simulink library "tof_lib"  (R2026a)
settings: Solver=VariableStepAuto
values from neighbouring files (symbols this model uses):
  fc_tofGain = Simulink.Parameter(1.00901);    fc_tofGain.CoderInfo.StorageClass      = 'ExportedGlobal'    [init_params.m]
  fc_tofIntercept = Simulink.Parameter(14.477);     fc_tofIntercept.CoderInfo.StorageClass = 'ExportedGlobal'    [init_params.m]
settings Model: Creator=Cyril Calo  LastModifiedBy=Cyril Calo

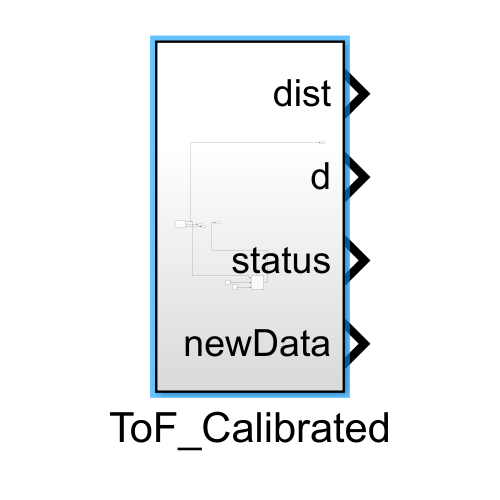
[thumbnail: Simulink's stored preview of the top-level diagram]
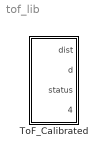
== system tof_lib ==
  ToF_Calibrated : Subsystem

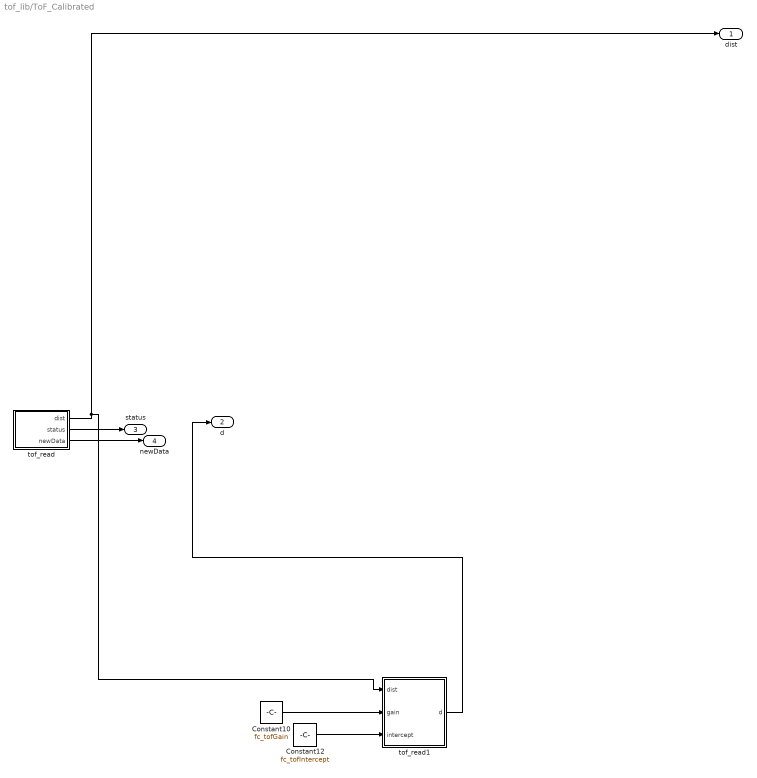
== system tof_lib/ToF_Calibrated ==
  Constant10 : Constant  Value=fc_tofGain
  Constant12 : Constant  Value=fc_tofIntercept
  tof_read : MATLAB Function  TreatAsAtomicUnit=on
  tof_read1 : MATLAB Function  TreatAsAtomicUnit=on
  dist : Outport
  d : Outport  Port=2
  status : Outport  Port=3
  newData : Outport  Port=4
  wires:
  tof_read/3(newData) -> newData/1
  tof_read/2(status) -> status/1
  Constant10/1 -> tof_read1/2(gain)
  Constant12/1 -> tof_read1/3(intercept)
  tof_read/1(dist) -> tof_read1/1(dist), dist/1
  tof_read1/1(d) -> d/1

== matlab function tof_lib/ToF_Calibrated/tof_read ==
  data: dist output; status output; newData output
function [dist, status, newData] = tof_read() %#codegen
coder.extrinsic('which', 'fileparts');
dist    = uint16(0);
status  = uint8(255);
newData = uint8(0);

persistent k started
if isempty(k)
    k = uint16(0);
    started = false;
end

if coder.target('Sfun')
    dist    = uint16(150) - mod(k, uint16(100));
    k       = k + uint16(1);
    status  = uint8(0);
    newData = uint8(1);
else
    srcDir = coder.const(fileparts(which('tof_wrapper.c')));
    coder.cinclude('tof_wrapper.h');
    coder.updateBuildInfo('addIncludePaths', srcDir);
    coder.updateBuildInfo('addSourcePaths',  srcDir);
    coder.updateBuildInfo('addSourceFiles', 'tof_wrapper.c');
    coder.updateBuildInfo('addSourceFiles', 'VL53L4CD_api.c');
    coder.updateBuildInfo('addSourceFiles', 'platform.c');

    if ~started
        coder.ceval('tof_init', int16(-26), uint16(200));
        started = true;
    end
    coder.ceval('tof_step', coder.wref(dist), coder.wref(status), coder.wref(newData));
end
end

== matlab function tof_lib/ToF_Calibrated/tof_read1 ==
  data: d output; dist input; gain input; intercept input
function d = tof_correct(dist, gain, intercept) %#codegen
% same formula as tofCorrect() in tof_cal.cpp: corrected = (raw - b) / m
if dist == 0
    d = 0;                        % no reading yet, pass through
else
    d = (double(dist) - intercept) / gain;
end
end
